simulink model "s_hover"  (Simulink 8.0)
settings: Solver=ode1  StartTime=0.0  StopTime=20  FixedStep=0.002  RelTol=1e-3
values from neighbouring files (symbols this model uses):
  CMD_RATE_LIMIT = 60 * pi/180    (= 1.0471975512)    [setup_lab_hover.m]
  K = lqr( A, B, Q, R )    [setup_lab_hover.m]
  K_AMP = 3    [setup_lab_hover.m]
  V_bias = 2.0    (= 2)    [setup_lab_hover.m]
  VMAX_AMP = 24    [setup_lab_hover.m]
  VMAX_DAC = 10    [setup_lab_hover.m]
  wcf = 2 * pi * 20    (= 125.663706144)    [setup_lab_hover.m]
  zetaf = 0.8    [setup_lab_hover.m]
undefined symbols (not defined in the file or in its folder): A, B, C, D
libraries: simulink_extras x5
settings Model: Creator=hpineros  LastModifiedBy=MLevis  ExtModeTrigDuration=10000
settings SolverCC: PositivePriorityOrder=on
settings DataIOCC: SignalLoggingSaveFormat=ModelDataLogs
settings OptimizationCC: InitFltsAndDblsToZero=on
settings DebuggingCC: SaveWithParameterizedLinksMsg=none  FcnCallInpInsideContextMsg=UseLocalSettings  StrictBusMsg=Warning
settings RTWCC: SystemTargetFile=quarc_windows.tlc  TemplateMakefile=quarc_default_tmf  Description=QuaRC Win32 Target  ProcessScript=quarc_windows_make_rtw_hook
settings STFCustomTargetCC: TargetFcnLib=ansi_tfl_tmw.mat  TargetPreCompLibLocation=C:\PROGRA~3\QUARC\lib\2012b\windows\release  CodeReplacementLibrary=ANSI_C  GeneratePreprocessorConditionals=Disable all  SystemTargetFile=quarc_windows.tlc
settings GRTTargetCC: TargetFcnLib=ansi_tfl_tmw.mat  TargetPreCompLibLocation=C:\PROGRA~3\QUARC\lib\2012b\windows\release  ParMdlRefBuildCompliant=off  CompOptLevelCompliant=off  ConcurrentExecutionCompliant=off  CombineOutputUpdateFcns=off  MatFileLogging=off  GRTInterface=on  ExtMode=on  ExtModeMexFile=quarc_comm

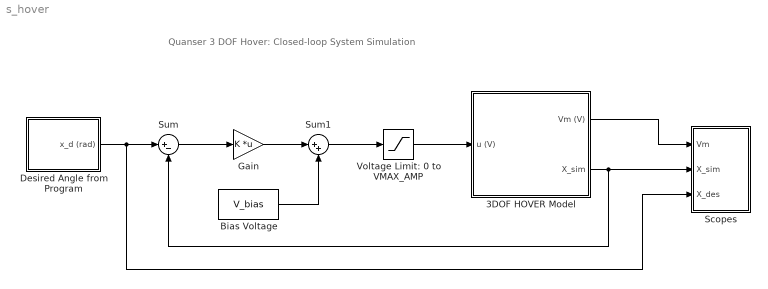
== system s_hover ==
  note: Quanser 3 DOF Hover:
      | Closed-loop System Simulation
  3DOF HOVER Model : Subsystem
  Bias Voltage : Constant  Value=V_bias
  Desired Angle from Program : Subsystem
  Gain : Gain  Gain=K  Multiplication=Matrix(K*u)
  Scopes : Subsystem
  Sum : Sum  Inputs=|+-
  Sum1 : Sum  Inputs=|++
  Voltage Limit: 0 to VMAX_AMP : Saturate  UpperLimit=VMAX_AMP  LowerLimit=0
  wires:
  Desired Angle from Program/1(x_d (rad)) -> Scopes/3(X_des), Sum/1
  Sum/1 -> Gain/1
  Gain/1 -> Sum1/1
  Bias Voltage/1 -> Sum1/2
  Sum1/1 -> Voltage Limit: 0 to VMAX_AMP/1
  Voltage Limit: 0 to VMAX_AMP/1 -> 3DOF HOVER Model/1(u (V))
  3DOF HOVER Model/1(Vm (V)) -> Scopes/1(Vm)
  3DOF HOVER Model/2(X_sim) -> Sum/2, Scopes/2(X_sim)

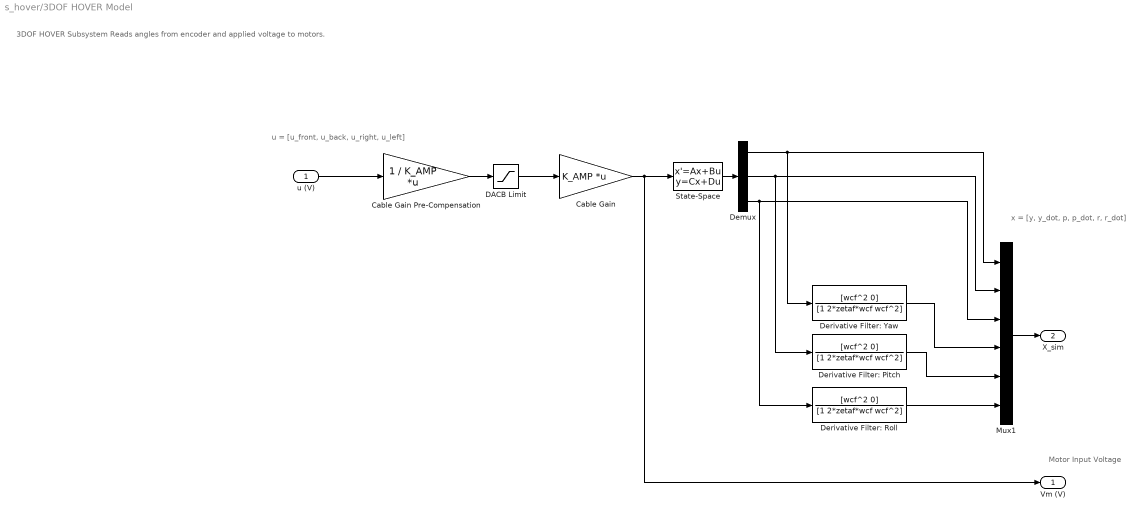
== system s_hover/3DOF HOVER Model ==
  note: 3DOF HOVER Subsystem
      | Reads angles from encoder and applied voltage to motors.
  note: Motor Input Voltage
  note: u = [u_front, u_back, u_right, u_left]
  note: x = [y, y_dot, p, p_dot, r, r_dot]
  u (V) : Inport
  Cable Gain : Gain  Gain=K_AMP  Multiplication=Matrix(K*u)  SaturateOnIntegerOverflow=on  OutDataTypeStr=Inherit: Same as input  ParamDataTypeStr=Inherit: Same as input
  Cable Gain Pre-Compensation : Gain  Gain=1 / K_AMP  Multiplication=Matrix(K*u)  SaturateOnIntegerOverflow=on  OutDataTypeStr=Inherit: Same as input  ParamDataTypeStr=Inherit: Same as input
  DACB Limit : Saturate  UpperLimit=VMAX_DAC  LowerLimit=-VMAX_DAC
  Demux : Demux  Outputs=3
  Derivative Filter: Pitch : TransferFcn  Numerator=[wcf^2 0]  Denominator=[1 2*zetaf*wcf wcf^2]
  Derivative Filter: Roll : TransferFcn  Numerator=[wcf^2 0]  Denominator=[1 2*zetaf*wcf wcf^2]
  Derivative Filter: Yaw : TransferFcn  Numerator=[wcf^2 0]  Denominator=[1 2*zetaf*wcf wcf^2]
  Mux1 : Mux  Inputs=6
  State-Space : StateSpace  A=A  B=B  C=C  D=D
  Vm (V) : Outport
  X_sim : Outport  Port=2
  wires:
  Demux/3 -> Derivative Filter: Roll/1, Mux1/3
  Demux/2 -> Derivative Filter: Pitch/1, Mux1/2
  Derivative Filter: Roll/1 -> Mux1/6
  Derivative Filter: Pitch/1 -> Mux1/5
  Derivative Filter: Yaw/1 -> Mux1/4
  Demux/1 -> Derivative Filter: Yaw/1, Mux1/1
  State-Space/1 -> Demux/1
  Mux1/1 -> X_sim/1
  Cable Gain/1 -> State-Space/1, Vm (V)/1
  DACB Limit/1 -> Cable Gain/1
  Cable Gain Pre-Compensation/1 -> DACB Limit/1
  u (V)/1 -> Cable Gain Pre-Compensation/1

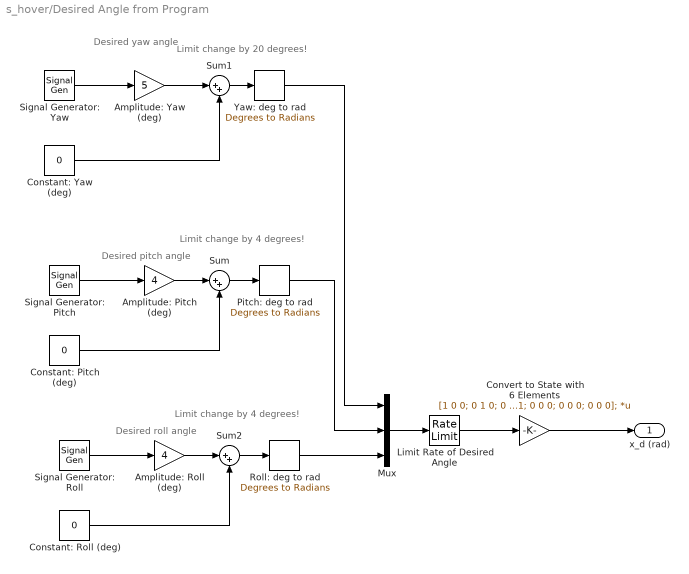
== system s_hover/Desired Angle from Program ==
  note: Limit change by
      | 4 degrees!
  note: Limit change by
      | 20 degrees!
  note: Limit change by
      | 4 degrees!
  note: Desired roll angle
  note: Desired pitch angle
  note: Desired yaw angle
  Amplitude: Pitch (deg) : Gain  Gain=4
  Amplitude: Roll (deg) : Gain  Gain=4
  Amplitude: Yaw (deg) : Gain  Gain=5
  Constant: Pitch (deg) : Constant  Value=0
  Constant: Roll (deg) : Constant  Value=0
  Constant: Yaw (deg) : Constant  Value=0
  Convert to State with 6 Elements : Gain  Gain=[1 0 0; 0 1 0; 0 0 1; 0 0 0; 0 0 0; 0 0 0];  Multiplication=Matrix(K*u)
  Limit Rate of Desired Angle : RateLimiter  RisingSlewLimit=CMD_RATE_LIMIT  FallingSlewLimit=-CMD_RATE_LIMIT
  Mux : Mux  Inputs=3
  Pitch: deg to rad : simulink_extras/Transformations/Degrees to Radians
  Roll: deg to rad : simulink_extras/Transformations/Degrees to Radians
  Signal Generator: Pitch : SignalGenerator  WaveForm=square  Frequency=0.1
  Signal Generator: Roll : SignalGenerator  WaveForm=square  Frequency=0.08
  Signal Generator: Yaw : SignalGenerator  WaveForm=square  Frequency=0.04
  Sum : Sum  Inputs=|++
  Sum1 : Sum  Inputs=|++
  Sum2 : Sum  Inputs=|++
  Yaw: deg to rad : simulink_extras/Transformations/Degrees to Radians
  x_d (rad) : Outport
  wires:
  Convert to State with 6 Elements/1 -> x_d (rad)/1
  Limit Rate of Desired Angle/1 -> Convert to State with 6 Elements/1
  Roll: deg to rad/1 -> Mux/3
  Pitch: deg to rad/1 -> Mux/2
  Yaw: deg to rad/1 -> Mux/1
  Sum2/1 -> Roll: deg to rad/1
  Signal Generator: Roll/1 -> Amplitude: Roll (deg)/1
  Amplitude: Roll (deg)/1 -> Sum2/1
  Constant: Roll (deg)/1 -> Sum2/2
  Sum/1 -> Pitch: deg to rad/1
  Signal Generator: Pitch/1 -> Amplitude: Pitch (deg)/1
  Amplitude: Pitch (deg)/1 -> Sum/1
  Constant: Pitch (deg)/1 -> Sum/2
  Sum1/1 -> Yaw: deg to rad/1
  Signal Generator: Yaw/1 -> Amplitude: Yaw (deg)/1
  Amplitude: Yaw (deg)/1 -> Sum1/1
  Constant: Yaw (deg)/1 -> Sum1/2
  Mux/1 -> Limit Rate of Desired Angle/1

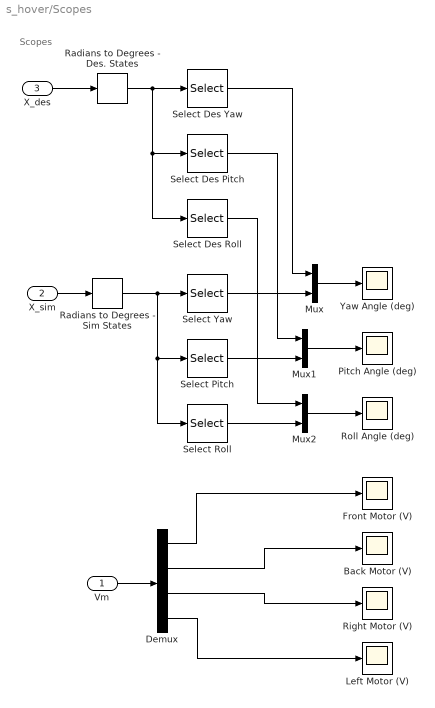
== system s_hover/Scopes ==
  note: Scopes
  Vm : Inport
  X_sim : Inport  Port=2
  X_des : Inport  Port=3
  Back Motor (V) : Scope
      settings: TimeRange=20  YMax=20  SaveName=data_Vb  MaxDataPoints=10000
  Demux : Demux
  Front Motor (V) : Scope
      settings: TimeRange=20  YMax=20  SaveName=data_Vf  MaxDataPoints=10000
  Left Motor (V) : Scope
      settings: TimeRange=20  YMax=20  SaveName=data_Vl  MaxDataPoints=10000
  Mux : Mux  Inputs=2
  Mux1 : Mux  Inputs=2
  Mux2 : Mux  Inputs=2
  Pitch Angle (deg) : Scope
      settings: TimeRange=20  SaveName=data_pitch  MaxDataPoints=10000
  Radians to Degrees - Des. States : simulink_extras/Transformations/Radians to Degrees
  Radians to Degrees - Sim States : simulink_extras/Transformations/Radians to Degrees
  Right Motor (V) : Scope
      settings: TimeRange=20  YMax=20  SaveName=data_Vr  MaxDataPoints=10000
  Roll Angle (deg) : Scope
      settings: TimeRange=20  SaveName=data_roll  MaxDataPoints=10000
  Select Des Pitch : Selector  InputPortWidth=6  IndexOptions=Index vector (dialog)  Indices=2  OutputSizes=1
  Select Des Roll : Selector  InputPortWidth=6  IndexOptions=Index vector (dialog)  Indices=3  OutputSizes=1
  Select Des Yaw : Selector  InputPortWidth=6  IndexOptions=Index vector (dialog)  Indices=1  OutputSizes=1
  Select Pitch : Selector  InputPortWidth=6  IndexOptions=Index vector (dialog)  Indices=2  OutputSizes=1
  Select Roll : Selector  InputPortWidth=6  IndexOptions=Index vector (dialog)  Indices=3  OutputSizes=1
  Select Yaw : Selector  InputPortWidth=6  IndexOptions=Index vector (dialog)  Indices=1  OutputSizes=1
  Yaw Angle (deg) : Scope
      settings: TimeRange=20  YMin=-6  YMax=6  SaveName=data_yaw  MaxDataPoints=10000
  wires:
  Select Des Roll/1 -> Mux2/1
  Select Des Pitch/1 -> Mux1/1
  Select Des Yaw/1 -> Mux/1
  Radians to Degrees - Des. States/1 -> Select Des Roll/1, Select Des Pitch/1, Select Des Yaw/1
  Select Roll/1 -> Mux2/2
  Select Pitch/1 -> Mux1/2
  Select Yaw/1 -> Mux/2
  Mux2/1 -> Roll Angle (deg)/1
  Radians to Degrees - Sim States/1 -> Select Roll/1, Select Pitch/1, Select Yaw/1
  Mux1/1 -> Pitch Angle (deg)/1
  Mux/1 -> Yaw Angle (deg)/1
  X_sim/1 -> Radians to Degrees - Sim States/1
  X_des/1 -> Radians to Degrees - Des. States/1
  Vm/1 -> Demux/1
  Demux/1 -> Front Motor (V)/1
  Demux/2 -> Back Motor (V)/1
  Demux/3 -> Right Motor (V)/1
  Demux/4 -> Left Motor (V)/1
